simulink model "hover_test_mdl"  (R2025a)
settings: Solver=VariableStepAuto  StartTime=0.0  StopTime=T_end  RelTol=1e-3
values from neighbouring files (symbols this model uses):
  K_AZ = 20    [rotation_demo.m]
  Kd = 4    [rotation_demo.m]
  Kp = 4    [rotation_demo.m]
  Ts = 0.05    [motor_test.m]    (also in rotation_demo.m)
  Z_REF = 0.5    [rotation_demo.m]
settings Model: Creator=maximeboulin  LastModifiedBy=maximeboulin

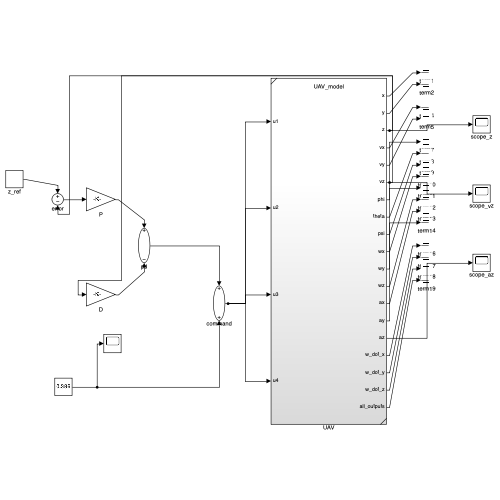
[thumbnail: Simulink's stored preview of the top-level diagram]
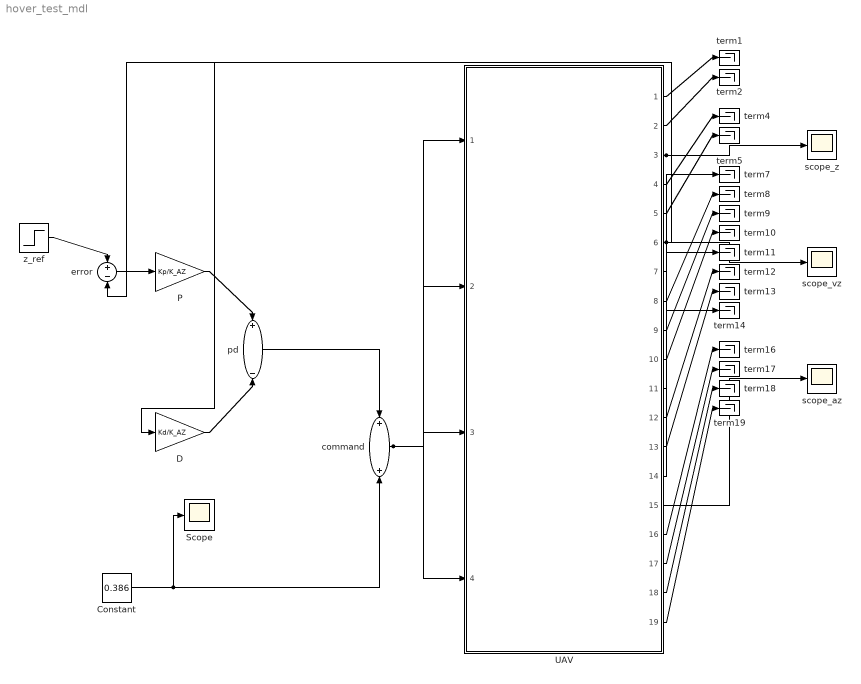
== system hover_test_mdl ==
  Constant : Constant  Value=0.386  SampleTime=0.05
  D : Gain  Gain=Kd/K_AZ
  P : Gain  Gain=Kp/K_AZ
  Scope : Scope
      settings: ActiveDisplayYMinimum=0.28600000000000003  ActiveDisplayYMaximum=0.486
  UAV : Subsystem  ReferencedSubsystem=UAV_model
  command : Sum
  error : Sum  Inputs=+-
  pd : Sum  Inputs=+-
  scope_az : Scope
  scope_vz : Scope
  scope_z : Scope
      settings: ActiveDisplayYMinimum=-0.62973466342741269  ActiveDisplayYMaximum=0.62572461082771325
  term{1..2,4..5,7..14,16..19} (16 alike) : Terminator
  z_ref : Step  After=Z_REF  SampleTime=Ts
  wires:
  UAV/3 -> scope_z/1, error/2
  UAV/6 -> scope_vz/1, D/1
  UAV/15 -> scope_az/1
  UAV/1 -> term1/1
  UAV/2 -> term2/1
  UAV/4 -> term4/1
  UAV/5 -> term5/1
  UAV/7 -> term7/1
  UAV/8 -> term8/1
  UAV/9 -> term9/1
  UAV/10 -> term10/1
  UAV/11 -> term11/1
  UAV/12 -> term12/1
  UAV/13 -> term13/1
  UAV/14 -> term14/1
  UAV/16 -> term16/1
  UAV/17 -> term17/1
  UAV/18 -> term18/1
  UAV/19 -> term19/1
  z_ref/1 -> error/1
  error/1 -> P/1
  P/1 -> pd/1
  D/1 -> pd/2
  Constant/1 -> Scope/1, command/2
  pd/1 -> command/1
  command/1 -> UAV/1, UAV/2, UAV/3, UAV/4
